simulink model "six_stepItext"  (R2024a)
settings: Solver=ode23t  StartTime=0.0  StopTime=10  MaxStep=1e-6  RelTol=1e-4
undefined symbols (not defined in the file): DiscIntNeverNeededParam
libraries: simulink x24, nesl_utility x13, ee_lib x6, fl_lib x6, eePwmGenerator x1
(part 2 of 2)

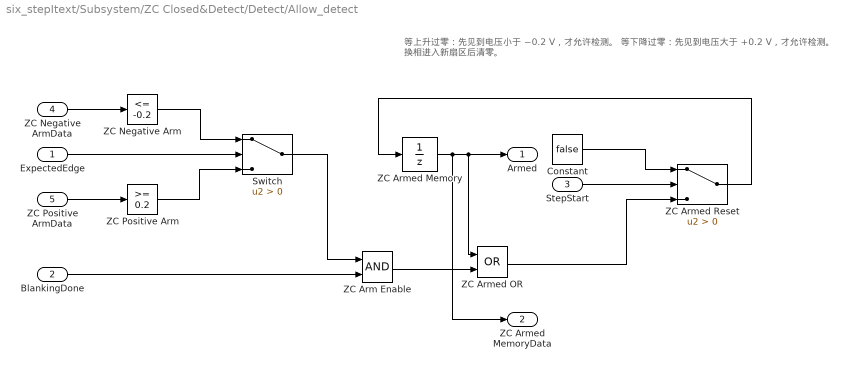
== system six_stepItext/Subsystem/ZC Closed&Detect/Detect/Allow_detect ==
  note: 等上升过零：先见到电压小于 −0.2 V，才允许检测。
      | 等下降过零：先见到电压大于 +0.2 V，才允许检测。
      | 换相进入新扇区后清零。
  ExpectedEdge : Inport
  BlankingDone : Inport  Port=2
  StepStart : Inport  Port=3
  ZC Negative ArmData : Inport  Port=4
  ZC Positive ArmData : Inport  Port=5
  Constant : Constant  Value=false
  Switch : Switch  Criteria=u2 > Threshold  SaturateOnIntegerOverflow=off  InputSameDT=off
  ZC Arm Enable : Logic  AllPortsSameDT=off  OutDataTypeStr=boolean
  ZC Armed Memory : UnitDelay  InitialCondition=false  SampleTime=10e-6  HasFrameUpgradeWarning=on
  ZC Armed OR : Logic  Operator=OR  AllPortsSameDT=off  OutDataTypeStr=boolean
  ZC Armed Reset : Switch  Criteria=u2 > Threshold  SaturateOnIntegerOverflow=off  InputSameDT=off
  ZC Negative Arm : simulink/Logic and Bit Operations/Compare To Constant  relop=<=  const=-0.2  OutDataTypeStr=boolean
  ZC Positive Arm : simulink/Logic and Bit Operations/Compare To Constant  relop=>=  const=0.2  OutDataTypeStr=boolean
  Armed : Outport
  ZC Armed MemoryData : Outport  Port=2
  wires:
  ZC Negative Arm/1 -> Switch/1
  ZC Positive Arm/1 -> Switch/3
  ExpectedEdge/1 -> Switch/2
  BlankingDone/1 -> ZC Arm Enable/2
  Switch/1 -> ZC Arm Enable/1
  ZC Arm Enable/1 -> ZC Armed OR/2
  ZC Armed Memory/1 -> ZC Armed MemoryData/1, Armed/1, ZC Armed OR/1
  Constant/1 -> ZC Armed Reset/1
  StepStart/1 -> ZC Armed Reset/2
  ZC Armed OR/1 -> ZC Armed Reset/3
  ZC Armed Reset/1 -> ZC Armed Memory/1
  ZC Negative ArmData/1 -> ZC Negative Arm/1
  ZC Positive ArmData/1 -> ZC Positive Arm/1

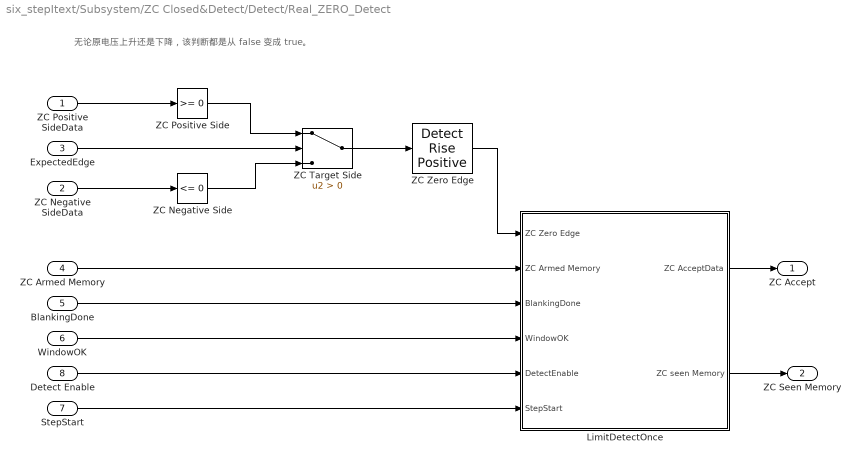
== system six_stepItext/Subsystem/ZC Closed&Detect/Detect/Real_ZERO_Detect ==
  note: 无论原电压上升还是下降，该判断都是从 false 变成 true。
  ZC Positive SideData : Inport
  ZC Negative SideData : Inport  Port=2
  ExpectedEdge : Inport  Port=3
  ZC Armed Memory : Inport  Port=4
  BlankingDone : Inport  Port=5
  WindowOK : Inport  Port=6
  StepStart : Inport  Port=7
  Detect Enable : Inport  Port=8
  LimitDetectOnce : Subsystem
  ZC Negative Side : simulink/Logic and Bit Operations/Compare To Constant  relop=<=  const=0  OutDataTypeStr=boolean
  ZC Positive Side : simulink/Logic and Bit Operations/Compare To Constant  relop=>=  const=0  OutDataTypeStr=boolean
  ZC Target Side : Switch  Criteria=u2 > Threshold  SaturateOnIntegerOverflow=off  InputSameDT=off
  ZC Zero Edge : simulink/Logic and Bit Operations/Detect Rise Positive  vinit=0  OutDataTypeStr=boolean
  ZC Accept : Outport
  ZC Seen Memory : Outport  Port=2
  wires:
  ZC Positive SideData/1 -> ZC Positive Side/1
  ZC Negative SideData/1 -> ZC Negative Side/1
  ZC Positive Side/1 -> ZC Target Side/1
  ZC Negative Side/1 -> ZC Target Side/3
  ExpectedEdge/1 -> ZC Target Side/2
  ZC Target Side/1 -> ZC Zero Edge/1
  ZC Armed Memory/1 -> LimitDetectOnce/2(ZC Armed Memory)
  ZC Zero Edge/1 -> LimitDetectOnce/1(ZC Zero Edge)
  LimitDetectOnce/1(ZC AcceptData) -> ZC Accept/1
  BlankingDone/1 -> LimitDetectOnce/3(BlankingDone)
  WindowOK/1 -> LimitDetectOnce/4(WindowOK)
  StepStart/1 -> LimitDetectOnce/6(StepStart)
  Detect Enable/1 -> LimitDetectOnce/5(DetectEnable)
  LimitDetectOnce/2(ZC seen Memory) -> ZC Seen Memory/1

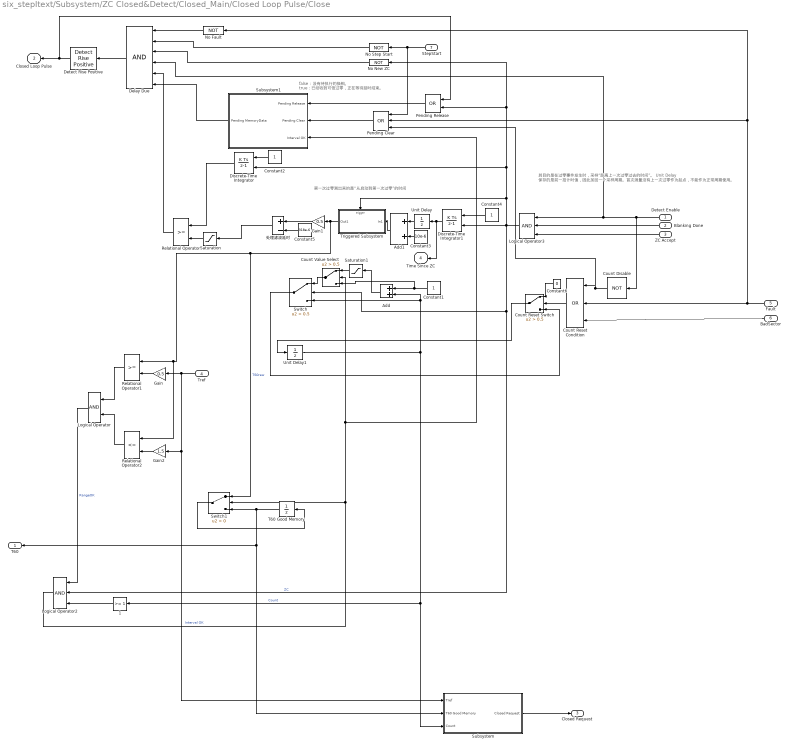
== system six_stepItext/Subsystem/ZC Closed&Detect/Closed_Main/Closed Loop Pulse/Close ==
  note: 其目的是在过零事件发生时，采样“距离上一次过零过去的时间”。 Unit Delay 保存的是前一拍计时值，因此加回一个采样周期。首次测量没有上一次过零作为起点，不能作为正常周期使用。
  note: 第一次过零测出来的是“从启动到第一次过零”的时间
  note: false：没有待执行的换相。
      | true：已经收到可信过零，正在等待延时结束。
  Detect Enable : Inport
  Blanking Done : Inport  Port=2
  ZC Accept : Inport  Port=3
  Tref : Inport  Port=4
  Fault : Inport  Port=5
  BadSector : Inport  Port=6
  StepStart : Inport  Port=7
  1 : simulink/Logic and Bit Operations/Compare To Constant  relop=>=  const=1  OutDataTypeStr=boolean
  Add : Sum
  Add1 : Sum
  Constant1 : Constant
  Constant2 : Constant
  Constant3 : Constant  Value=10e-6
  Constant4 : Constant
  Constant5 : Constant  Value=318e-6
  Constant6 : Constant  Value=0
  Count Disable : Logic  Operator=NOT  Inputs=3  AllPortsSameDT=off  OutDataTypeStr=boolean
  Count Reset Condition : Logic  Operator=OR  Inputs=3  AllPortsSameDT=off  OutDataTypeStr=boolean
  Count Reset Switch : Switch  Criteria=u2 > Threshold  Threshold=0.5  SaturateOnIntegerOverflow=off  InputSameDT=off
  Count Value Select : Switch  Criteria=u2 > Threshold  Threshold=0.5  SaturateOnIntegerOverflow=off  InputSameDT=off
  Delay Due : Logic  Inputs=6  AllPortsSameDT=off  OutDataTypeStr=boolean
  Detect Rise Positive : simulink/Logic and Bit Operations/Detect Rise Positive  vinit=0  OutDataTypeStr=boolean
  Discrete-Time Integrator : DiscreteIntegrator  ExternalReset=rising  SampleTime=10e-6  ICPrevOutput=DiscIntNeverNeededParam  ICPrevScaledInput=DiscIntNeverNeededParam
  Discrete-Time Integrator1 : DiscreteIntegrator  ExternalReset=rising  SampleTime=10e-6  ICPrevOutput=DiscIntNeverNeededParam  ICPrevScaledInput=DiscIntNeverNeededParam
  Gain : Gain  Gain=0.5
  Gain1 : Gain  Gain=0.5
  Gain2 : Gain  Gain=1.5
  Logical Operator : Logic  AllPortsSameDT=off  OutDataTypeStr=boolean
  Logical Operator2 : Logic  Inputs=3  AllPortsSameDT=off  OutDataTypeStr=boolean
  Logical Operator3 : Logic  Inputs=3  AllPortsSameDT=off  OutDataTypeStr=boolean
  No Fault : Logic  Operator=NOT  Inputs=3  AllPortsSameDT=off  OutDataTypeStr=boolean
  No New ZC : Logic  Operator=NOT  Inputs=3  AllPortsSameDT=off  OutDataTypeStr=boolean
  No Step Start : Logic  Operator=NOT  Inputs=3  AllPortsSameDT=off  OutDataTypeStr=boolean
  Pending Clear : Logic  Operator=OR  Inputs=3  AllPortsSameDT=off  OutDataTypeStr=boolean
  Pending Release : Logic  Operator=OR  AllPortsSameDT=off  OutDataTypeStr=boolean
  Relational Operator : RelationalOperator  OutDataTypeStr=boolean  RndMeth=Simplest  InputSameDT=off
  Relational Operator1 : RelationalOperator  OutDataTypeStr=boolean  RndMeth=Simplest  InputSameDT=off
  Relational Operator2 : RelationalOperator  Operator=<=  OutDataTypeStr=boolean  RndMeth=Simplest  InputSameDT=off
  Saturation : Saturate  UpperLimit=0.05  LowerLimit=10e-6
  Saturation1 : Saturate  UpperLimit=10  LowerLimit=0
  Subsystem : Subsystem
  Subsystem1 : Subsystem
  Switch : Switch  Criteria=u2 > Threshold  Threshold=0.5  SaturateOnIntegerOverflow=off  InputSameDT=off
  Switch1 : Switch  Criteria=u2 > Threshold  SaturateOnIntegerOverflow=off  InputSameDT=off
  T60 Good Memory : UnitDelay  InitialCondition=0.02  SampleTime=10e-6  HasFrameUpgradeWarning=on
  Triggered Subsystem : Subsystem  TreatAsAtomicUnit=on
  Unit Delay : UnitDelay  SampleTime=10e-6  HasFrameUpgradeWarning=on
  Unit Delay1 : UnitDelay  SampleTime=10e-6  HasFrameUpgradeWarning=on
  处理滤波延时 : Sum  Inputs=+-
  T60 : Outport
  Closed Loop Pulse : Outport  Port=2
  Closed Request : Outport  Port=3
  Time Since ZC : Outport  Port=4
  wires:
  Gain1/1 -> 处理滤波延时/1
  Triggered Subsystem/1(Out1) -> Switch1/1, Relational Operator2/1, Relational Operator1/1, Gain1/1  "T60raw"
  Detect Enable/1 -> Delay Due/4, Logical Operator3/1, Count Disable/1
  Constant4/1 -> Discrete-Time Integrator1/1
  Discrete-Time Integrator1/1 -> Time Since ZC/1, Unit Delay/1
  Logical Operator3/1 -> No New ZC/1, Pending Release/2, Discrete-Time Integrator/2, Triggered Subsystem/Trigger, Logical Operator2/2, Switch/2, Discrete-Time Integrator1/2  "ZC"
  Constant5/1 -> 处理滤波延时/2
  ZC Accept/1 -> Logical Operator3/3
  Blanking Done/1 -> Logical Operator3/2
  处理滤波延时/1 -> Saturation/1
  Constant2/1 -> Discrete-Time Integrator/1
  Saturation/1 -> Relational Operator/2
  Discrete-Time Integrator/1 -> Relational Operator/1
  Relational Operator/1 -> Delay Due/5
  Constant1/1 -> Count Value Select/3, Add/1
  Add/1 -> Saturation1/1
  Unit Delay1/1 -> 1/1, Subsystem/3(Count), Switch/3, Add/2  "Count"
  Relational Operator1/1 -> Logical Operator/1
  Relational Operator2/1 -> Logical Operator/2
  Logical Operator/1 -> Logical Operator2/1  "RangeOK"
  Add1/1 -> Triggered Subsystem/1(In1)
  Unit Delay/1 -> Add1/1
  Constant3/1 -> Add1/2
  Tref/1 -> Subsystem/1(Tref), Gain2/1, Gain/1
  Gain/1 -> Relational Operator1/2
  Gain2/1 -> Relational Operator2/2
  T60 Good Memory/1 -> Subsystem/2(T60 Good Memory), T60/1, Switch1/3
  Switch1/1 -> T60 Good Memory/1
  1/1 -> Logical Operator2/3
  Logical Operator2/1 -> Switch1/2, Subsystem1/3(Interval OK), Count Value Select/2  "Interval OK"
  Saturation1/1 -> Count Value Select/1
  Count Value Select/1 -> Switch/1
  Count Disable/1 -> Pending Clear/3, Count Reset Condition/1
  Fault/1 -> Pending Clear/2, No Fault/1, Count Reset Condition/2
  BadSector/1 -> Count Reset Condition/3
  Constant6/1 -> Count Reset Switch/1
  Count Reset Condition/1 -> Count Reset Switch/2
  Count Reset Switch/1 -> Unit Delay1/1
  Switch/1 -> Count Reset Switch/3
  Subsystem/1(Closed Request) -> Closed Request/1
  StepStart/1 -> Pending Clear/1, No Step Start/1
  No Fault/1 -> Delay Due/1
  No Step Start/1 -> Delay Due/2
  No New ZC/1 -> Delay Due/3
  Delay Due/1 -> Detect Rise Positive/1
  Subsystem1/1(Pending MemoryData) -> Delay Due/6
  Detect Rise Positive/1 -> Pending Release/1, Closed Loop Pulse/1
  Pending Release/1 -> Subsystem1/1(Pending Release)
  Pending Clear/1 -> Subsystem1/2(Pending Clear)

== system six_stepItext/Subsystem/ZC Closed&Detect/Detect/Real_ZERO_Detect/LimitDetectOnce ==
  ZC Zero Edge : Inport
  ZC Armed Memory : Inport  Port=2
  BlankingDone : Inport  Port=3
  WindowOK : Inport  Port=4
  DetectEnable : Inport  Port=5
  StepStart : Inport  Port=6
  Constant : Constant  Value=false
  ZC Accept : Logic  Inputs=6  AllPortsSameDT=off  OutDataTypeStr=boolean
  ZC Not Seen : Logic  Operator=NOT  AllPortsSameDT=off  OutDataTypeStr=boolean
  ZC Seen Memory : UnitDelay  InitialCondition=false  SampleTime=10e-6  HasFrameUpgradeWarning=on
  ZC Seen OR : Logic  Operator=OR  AllPortsSameDT=off  OutDataTypeStr=boolean
  ZC Seen Reset : Switch  Criteria=u2 > Threshold  SaturateOnIntegerOverflow=off  InputSameDT=off
  ZC AcceptData : Outport
  ZC seen Memory : Outport  Port=2
  wires:
  ZC Seen Memory/1 -> ZC seen Memory/1, ZC Seen OR/1, ZC Not Seen/1
  ZC Accept/1 -> ZC AcceptData/1, ZC Seen OR/2
  Constant/1 -> ZC Seen Reset/1
  StepStart/1 -> ZC Seen Reset/2
  ZC Seen OR/1 -> ZC Seen Reset/3
  ZC Seen Reset/1 -> ZC Seen Memory/1
  ZC Not Seen/1 -> ZC Accept/1
  ZC Zero Edge/1 -> ZC Accept/2
  WindowOK/1 -> ZC Accept/3
  ZC Armed Memory/1 -> ZC Accept/4
  BlankingDone/1 -> ZC Accept/5
  DetectEnable/1 -> ZC Accept/6

== system six_stepItext/Subsystem/ZC Closed&Detect/Closed_Main/Closed Loop Pulse/Close/Subsystem ==
  Tref : Inport
  T60 Good Memory : Inport  Port=2
  Count : Inport  Port=3
  Closed Request Ready : Logic  AllPortsSameDT=off  OutDataTypeStr=boolean
  Compare To Constant : simulink/Logic and Bit Operations/Compare To Constant  relop=>=  const=10  OutDataTypeStr=boolean
  Period Difference : Sum  Inputs=+-
  Period Difference Abs : Abs  SaturateOnIntegerOverflow=off
  Period Match : RelationalOperator  Operator=<=  OutDataTypeStr=boolean  RndMeth=Simplest  InputSameDT=off
  Period Tolerance : Gain  Gain=0.15
  Scope : Scope
  Closed Request : Outport
  wires:
  T60 Good Memory/1 -> Period Difference/1
  Period Match/1 -> Closed Request Ready/2
  Period Difference/1 -> Period Difference Abs/1
  Tref/1 -> Period Difference/2, Period Tolerance/1
  Period Difference Abs/1 -> Period Match/1
  Period Tolerance/1 -> Period Match/2
  Count/1 -> Compare To Constant/1
  Compare To Constant/1 -> Closed Request Ready/1
  Closed Request Ready/1 -> Scope/1, Closed Request/1

== system six_stepItext/Subsystem/ZC Closed&Detect/Closed_Main/Closed Loop Pulse/Close/Subsystem1 ==
  note: 换相已经执行，或者来了新的但不可信的过零：取消旧任务。
      | 新过零及间隔可信：安排新任务。
      | 故障、进入新扇区或检测禁用：强制取消任务。
  Pending Release : Inport
  Pending Clear : Inport  Port=2
  Interval OK : Inport  Port=3
  Constant : Constant  Value=0  OutDataTypeStr=boolean
  Constant1 : Constant  OutDataTypeStr=boolean
  Constant2 : Constant  Value=0  OutDataTypeStr=boolean
  Pending Arm Switch : Switch  Criteria=u2 > Threshold  Threshold=0.5  SaturateOnIntegerOverflow=off  InputSameDT=off
  Pending Memory : UnitDelay  InitialCondition=false  SampleTime=10e-6  HasFrameUpgradeWarning=on
  Pending Release Switch : Switch  Criteria=u2 > Threshold  Threshold=0.5  SaturateOnIntegerOverflow=off  InputSameDT=off
  Pending Reset Switch : Switch  Criteria=u2 > Threshold  Threshold=0.5  SaturateOnIntegerOverflow=off  InputSameDT=off
  Pending MemoryData : Outport
  wires:
  Pending Release/1 -> Pending Release Switch/2
  Pending Memory/1 -> Pending MemoryData/1, Pending Release Switch/3
  Constant/1 -> Pending Release Switch/1
  Constant1/1 -> Pending Arm Switch/1
  Interval OK/1 -> Pending Arm Switch/2
  Pending Release Switch/1 -> Pending Arm Switch/3
  Constant2/1 -> Pending Reset Switch/1
  Pending Clear/1 -> Pending Reset Switch/2
  Pending Arm Switch/1 -> Pending Reset Switch/3
  Pending Reset Switch/1 -> Pending Memory/1

== system six_stepItext/Subsystem/ZC Closed&Detect/Closed_Main/Closed Loop Pulse/Close/Triggered Subsystem ==
  In1 : Inport
  Trigger : TriggerPort  VariantControl=(inherit)
  Out1 : Outport
  wires:
  In1/1 -> Out1/1
